simulink model "ZT_VehCtrl_18B_CAN"  (R2018b)
settings: Solver=FixedStepAuto  StartTime=0.0  StopTime=inf  FixedStep=0.005  RelTol=1e-3
InitFcn:
  | mbd_mpc_consistency_checks(bdroot(gcs));
values from neighbouring files (symbols this model uses):
  BatoverTempTh = single(80)    [VCU_INIT.m]
  BRS_PwrValid = single(5)    [VCU_INIT.m]
  BRSEnSpdTh1 = single(10)    [VCU_INIT.m]
  BRSEnSpdTh2 = single(20)    [VCU_INIT.m]
  MCUTempAlarmTh = single (60)    [VCU_INIT.m]
  mps2kmh = single(3.6)    [VCU_INIT.m]
  MtrPwrFac = single(1/9550)    [VCU_INIT.m]
  MtrTempAlarmTh = single (50)    [VCU_INIT.m]
  Padle1Signal1_Th = [PadleSignal1_min,PadleSignal1_max]    [VCU_INIT.m]
  Padle1Signal2_Th = [PadleSignal2_min,PadleSignal2_max]    [VCU_INIT.m]
  PadleSignal1_max = 3.84    [VCU_INIT.m]
  PadleSignal1_min = 0.75    [VCU_INIT.m]
  PadleSignal2_max = 1.92    [VCU_INIT.m]
  PadleSignal2_min = 0.375    [VCU_INIT.m]
  PadleValid = 0.05    [VCU_INIT.m]
  PwrLimFactor = single(0.5)    [VCU_INIT.m]
  Ratio = single(1)    [VCU_INIT.m]
  rpm2mps = single(2*pi/60 * WhlRadius/Ratio)    [VCU_INIT.m]
  SOCLowTh = single(20)    [VCU_INIT.m]
  VehPwrBackwardMax = VehPwrMax * single(0.3)    [VCU_INIT.m]
  VehPwrMax = single(MtrPwrMax * 4)    [VCU_INIT.m]
  VehTrqBackwardMax = VehTrqMax * single(0.3)    [VCU_INIT.m]
  VehTrqMax = single(MtrTrqMax * Ratio *4)    [VCU_INIT.m]
  WhlRadius = single(1)    [VCU_INIT.m]
undefined symbols (not defined in the file or in its folder): Delay_Charge, Delay_Discharge, fifo_0_vect, fifo_1_vect, LQFP, pts1_fifo_0_vect, pts1_fifo_1_vect, pts2_fifo_0_vect, pts2_fifo_1_vect, pts3_fifo_0_vect, pts3_fifo_1_vect, pts4_fifo_0_vect, pts4_fifo_1_vect
libraries: mbd_mpc574x_ec_toolbox x157, canmsglib x74, simulink x38
(part 6 of 12)

== system ZT_VehCtrl_18B_CAN/SigIn/CAN0 /BRS2VCU1 ==
  ID : Inport
  Data : Inport  Port=2
  length : Inport  Port=3
  timestamp : Inport  Port=4
  Switch Case : SwitchCase  CaseConditions={hex2dec('18FE25E4')}  ShowDefaultCase=off
  UNPACK : Subsystem  TreatAsAtomicUnit=on
  Message : Outport
  wires:
  Switch Case/1 -> UNPACK/Action
  ID/1 -> UNPACK/1(ID), Switch Case/1
  Data/1 -> UNPACK/2(data)
  timestamp/1 -> UNPACK/4(timestamp)
  length/1 -> UNPACK/3(length)
  UNPACK/1(Message) -> Message/1

== system ZT_VehCtrl_18B_CAN/SigIn/CAN0 /BRS2VCU2 ==
  ID : Inport
  Data : Inport  Port=2
  length : Inport  Port=3
  timestamp : Inport  Port=4
  Switch Case : SwitchCase  CaseConditions={hex2dec('18FE26E4')}  ShowDefaultCase=off
  UNPACK : Subsystem  TreatAsAtomicUnit=on
  Message : Outport
  wires:
  UNPACK/1(Message) -> Message/1
  length/1 -> UNPACK/3(length)
  timestamp/1 -> UNPACK/4(timestamp)
  Data/1 -> UNPACK/2(data)
  ID/1 -> Switch Case/1, UNPACK/1(ID)
  Switch Case/1 -> UNPACK/Action

== system ZT_VehCtrl_18B_CAN/SigIn/CAN0 /BRS2VCU3 ==
  ID : Inport
  Data : Inport  Port=2
  length : Inport  Port=3
  timestamp : Inport  Port=4
  Switch Case : SwitchCase  CaseConditions={hex2dec('18FE27E4')}  ShowDefaultCase=off
  UNPACK : Subsystem  TreatAsAtomicUnit=on
  Message : Outport
  wires:
  Switch Case/1 -> UNPACK/Action
  ID/1 -> UNPACK/1(ID), Switch Case/1
  Data/1 -> UNPACK/2(data)
  timestamp/1 -> UNPACK/4(timestamp)
  length/1 -> UNPACK/3(length)
  UNPACK/1(Message) -> Message/1

== system ZT_VehCtrl_18B_CAN/SigIn/CAN0 /OBC_Charger Status ==
  ID : Inport
  Data : Inport  Port=2
  length : Inport  Port=3
  timestamp : Inport  Port=4
  Switch Case : SwitchCase  CaseConditions={hex2dec('220')}  ShowDefaultCase=off
  UNPACK : Subsystem  TreatAsAtomicUnit=on
  Message : Outport
  wires:
  Switch Case/1 -> UNPACK/Action
  ID/1 -> UNPACK/1(ID), Switch Case/1
  Data/1 -> UNPACK/2(data)
  timestamp/1 -> UNPACK/4(timestamp)
  length/1 -> UNPACK/3(length)
  UNPACK/1(Message) -> Message/1

== system ZT_VehCtrl_18B_CAN/SigIn/CAN0 /PDU_RelaySts ==
  ID : Inport
  Data : Inport  Port=2
  length : Inport  Port=3
  timestamp : Inport  Port=4
  Switch Case : SwitchCase  CaseConditions={hex2dec('18FF2BC8')}  ShowDefaultCase=off
  UNPACK : Subsystem  TreatAsAtomicUnit=on
  Message : Outport
  wires:
  UNPACK/1(Message) -> Message/1
  length/1 -> UNPACK/3(length)
  timestamp/1 -> UNPACK/4(timestamp)
  Data/1 -> UNPACK/2(data)
  ID/1 -> Switch Case/1, UNPACK/1(ID)
  Switch Case/1 -> UNPACK/Action

== system ZT_VehCtrl_18B_CAN/SigIn/CAN0 /TMS2VCU ==
  ID : Inport
  Data : Inport  Port=2
  length : Inport  Port=3
  timestamp : Inport  Port=4
  Switch Case : SwitchCase  CaseConditions={hex2dec('18FFF346')}  ShowDefaultCase=off
  UNPACK : Subsystem  TreatAsAtomicUnit=on
  Message : Outport
  wires:
  UNPACK/1(Message) -> Message/1
  length/1 -> UNPACK/3(length)
  timestamp/1 -> UNPACK/4(timestamp)
  Data/1 -> UNPACK/2(data)
  ID/1 -> Switch Case/1, UNPACK/1(ID)
  Switch Case/1 -> UNPACK/Action

== system ZT_VehCtrl_18B_CAN/SigIn/CAN1/DCDC1_1 ==
  ID : Inport
  Data : Inport  Port=2
  length : Inport  Port=3
  timestamp : Inport  Port=4
  Switch Case : SwitchCase  CaseConditions={hex2dec('1800D08F')}  ShowDefaultCase=off
  UNPACK : Subsystem  TreatAsAtomicUnit=on
  Message : Outport
  wires:
  UNPACK/1(Message) -> Message/1
  length/1 -> UNPACK/3(length)
  timestamp/1 -> UNPACK/4(timestamp)
  Data/1 -> UNPACK/2(data)
  ID/1 -> Switch Case/1, UNPACK/1(ID)
  Switch Case/1 -> UNPACK/Action

== system ZT_VehCtrl_18B_CAN/SigIn/CAN1/DCDC1_2 ==
  ID : Inport
  Data : Inport  Port=2
  length : Inport  Port=3
  timestamp : Inport  Port=4
  Switch Case : SwitchCase  CaseConditions={hex2dec('1801D08F')}  ShowDefaultCase=off
  UNPACK : Subsystem  TreatAsAtomicUnit=on
  Message : Outport
  wires:
  Switch Case/1 -> UNPACK/Action
  ID/1 -> UNPACK/1(ID), Switch Case/1
  Data/1 -> UNPACK/2(data)
  timestamp/1 -> UNPACK/4(timestamp)
  length/1 -> UNPACK/3(length)
  UNPACK/1(Message) -> Message/1

== system ZT_VehCtrl_18B_CAN/SigIn/CAN1/HVC1_LV ==
  ID : Inport
  Data : Inport  Port=2
  length : Inport  Port=3
  timestamp : Inport  Port=4
  Switch Case : SwitchCase  CaseConditions={hex2dec('180105A1')}  ShowDefaultCase=off
  UNPACK : Subsystem  TreatAsAtomicUnit=on
  Message : Outport
  wires:
  Switch Case/1 -> UNPACK/Action
  ID/1 -> UNPACK/1(ID), Switch Case/1
  Data/1 -> UNPACK/2(data)
  timestamp/1 -> UNPACK/4(timestamp)
  length/1 -> UNPACK/3(length)
  UNPACK/1(Message) -> Message/1

== system ZT_VehCtrl_18B_CAN/SigIn/CAN1/HVC3_Temp ==
  ID : Inport
  Data : Inport  Port=2
  length : Inport  Port=3
  timestamp : Inport  Port=4
  Switch Case : SwitchCase  CaseConditions={hex2dec('180305A1')}  ShowDefaultCase=off
  UNPACK : Subsystem  TreatAsAtomicUnit=on
  Message : Outport
  wires:
  UNPACK/1(Message) -> Message/1
  length/1 -> UNPACK/3(length)
  timestamp/1 -> UNPACK/4(timestamp)
  Data/1 -> UNPACK/2(data)
  ID/1 -> Switch Case/1, UNPACK/1(ID)
  Switch Case/1 -> UNPACK/Action

== system ZT_VehCtrl_18B_CAN/SigIn/CAN1/HVC4_RlySt ==
  ID : Inport
  Data : Inport  Port=2
  length : Inport  Port=3
  timestamp : Inport  Port=4
  Switch Case : SwitchCase  CaseConditions={hex2dec('180405A1')}  ShowDefaultCase=off
  UNPACK : Subsystem  TreatAsAtomicUnit=on
  Message : Outport
  wires:
  Switch Case/1 -> UNPACK/Action
  ID/1 -> UNPACK/1(ID), Switch Case/1
  Data/1 -> UNPACK/2(data)
  timestamp/1 -> UNPACK/4(timestamp)
  length/1 -> UNPACK/3(length)
  UNPACK/1(Message) -> Message/1

== system ZT_VehCtrl_18B_CAN/SigIn/CAN1/HVC7_HV1 ==
  ID : Inport
  Data : Inport  Port=2
  length : Inport  Port=3
  timestamp : Inport  Port=4
  Switch Case : SwitchCase  CaseConditions={hex2dec('180705A1')}  ShowDefaultCase=off
  UNPACK : Subsystem  TreatAsAtomicUnit=on
  Message : Outport
  wires:
  UNPACK/1(Message) -> Message/1
  length/1 -> UNPACK/3(length)
  timestamp/1 -> UNPACK/4(timestamp)
  Data/1 -> UNPACK/2(data)
  ID/1 -> Switch Case/1, UNPACK/1(ID)
  Switch Case/1 -> UNPACK/Action

== system ZT_VehCtrl_18B_CAN/SigIn/CAN1/ISG MCU STATUS 1 ==
  ID : Inport
  Data : Inport  Port=2
  length : Inport  Port=3
  timestamp : Inport  Port=4
  Switch Case : SwitchCase  CaseConditions={hex2dec('CFF0006')}  ShowDefaultCase=off
  UNPACK : Subsystem  TreatAsAtomicUnit=on
  Message : Outport
  wires:
  Switch Case/1 -> UNPACK/Action
  ID/1 -> UNPACK/1(ID), Switch Case/1
  Data/1 -> UNPACK/2(data)
  timestamp/1 -> UNPACK/4(timestamp)
  length/1 -> UNPACK/3(length)
  UNPACK/1("Message ") -> Message/1

== system ZT_VehCtrl_18B_CAN/SigIn/CAN1/ISG MCU STATUS 2 ==
  ID : Inport
  Data : Inport  Port=2
  length : Inport  Port=3
  timestamp : Inport  Port=4
  Switch Case : SwitchCase  CaseConditions={hex2dec('CFF0106')}  ShowDefaultCase=off
  UNPACK : Subsystem  TreatAsAtomicUnit=on
  Message : Outport
  wires:
  UNPACK/1(Message1) -> Message/1
  length/1 -> UNPACK/3(length)
  timestamp/1 -> UNPACK/4(timestamp)
  Data/1 -> UNPACK/2(data)
  ID/1 -> Switch Case/1, UNPACK/1(ID)
  Switch Case/1 -> UNPACK/Action

== system ZT_VehCtrl_18B_CAN/SigIn/CAN1/ISG MCU STATUS 3 ==
  ID : Inport
  Data : Inport  Port=2
  length : Inport  Port=3
  timestamp : Inport  Port=4
  Switch Case : SwitchCase  CaseConditions={hex2dec('CFF0206')}  ShowDefaultCase=off
  UNPACK : Subsystem  TreatAsAtomicUnit=on
  Message : Outport
  wires:
  Switch Case/1 -> UNPACK/Action
  ID/1 -> UNPACK/1(ID), Switch Case/1
  Data/1 -> UNPACK/2(data)
  timestamp/1 -> UNPACK/4(timestamp)
  length/1 -> UNPACK/3(length)
  UNPACK/1(Message) -> Message/1

== system ZT_VehCtrl_18B_CAN/SigIn/CAN1/MCU1Msg1 ==
  ID : Inport
  Data : Inport  Port=2
  length : Inport  Port=3
  timestamp : Inport  Port=4
  Switch Case : SwitchCase  CaseConditions={hex2dec('1836D0EF')}  ShowDefaultCase=off
  UNPACK : Subsystem  TreatAsAtomicUnit=on
  Message : Outport
  wires:
  UNPACK/1(Message) -> Message/1
  length/1 -> UNPACK/3(length)
  timestamp/1 -> UNPACK/4(timestamp)
  Data/1 -> UNPACK/2(data)
  ID/1 -> Switch Case/1, UNPACK/1(ID)
  Switch Case/1 -> UNPACK/Action

== system ZT_VehCtrl_18B_CAN/SigIn/CAN1/MCU1Msg2 ==
  ID : Inport
  Data : Inport  Port=2
  length : Inport  Port=3
  timestamp : Inport  Port=4
  Switch Case : SwitchCase  CaseConditions={hex2dec('1837D0EF')}  ShowDefaultCase=off
  UNPACK : Subsystem  TreatAsAtomicUnit=on
  Message : Outport
  wires:
  Switch Case/1 -> UNPACK/Action
  ID/1 -> UNPACK/1(ID), Switch Case/1
  Data/1 -> UNPACK/2(data)
  timestamp/1 -> UNPACK/4(timestamp)
  length/1 -> UNPACK/3(length)
  UNPACK/1(Message) -> Message/1

== system ZT_VehCtrl_18B_CAN/SigIn/CAN1/MCU1Msg3 ==
  ID : Inport
  Data : Inport  Port=2
  length : Inport  Port=3
  timestamp : Inport  Port=4
  Switch Case : SwitchCase  CaseConditions={hex2dec('1838D0EF')}  ShowDefaultCase=off
  UNPACK : Subsystem  TreatAsAtomicUnit=on
  Message : Outport
  wires:
  UNPACK/1(Message) -> Message/1
  length/1 -> UNPACK/3(length)
  timestamp/1 -> UNPACK/4(timestamp)
  Data/1 -> UNPACK/2(data)
  ID/1 -> Switch Case/1, UNPACK/1(ID)
  Switch Case/1 -> UNPACK/Action

== system ZT_VehCtrl_18B_CAN/SigIn/CAN1/MCU2Msg1 ==
  ID : Inport
  Data : Inport  Port=2
  length : Inport  Port=3
  timestamp : Inport  Port=4
  Switch Case : SwitchCase  CaseConditions={hex2dec('1836D0F1')}  ShowDefaultCase=off
  UNPACK : Subsystem  TreatAsAtomicUnit=on
  Message : Outport
  wires:
  Switch Case/1 -> UNPACK/Action
  ID/1 -> UNPACK/1(ID), Switch Case/1
  Data/1 -> UNPACK/2(data)
  timestamp/1 -> UNPACK/4(timestamp)
  length/1 -> UNPACK/3(length)
  UNPACK/1(Message) -> Message/1

== system ZT_VehCtrl_18B_CAN/SigIn/CAN1/MCU2Msg2 ==
  ID : Inport
  Data : Inport  Port=2
  length : Inport  Port=3
  timestamp : Inport  Port=4
  Switch Case : SwitchCase  CaseConditions={hex2dec('1837D0F1')}  ShowDefaultCase=off
  UNPACK : Subsystem  TreatAsAtomicUnit=on
  Message : Outport
  wires:
  UNPACK/1(Message) -> Message/1
  length/1 -> UNPACK/3(length)
  timestamp/1 -> UNPACK/4(timestamp)
  Data/1 -> UNPACK/2(data)
  ID/1 -> Switch Case/1, UNPACK/1(ID)
  Switch Case/1 -> UNPACK/Action

== system ZT_VehCtrl_18B_CAN/SigIn/CAN1/MCU2Msg3 ==
  ID : Inport
  Data : Inport  Port=2
  length : Inport  Port=3
  timestamp : Inport  Port=4
  Switch Case : SwitchCase  CaseConditions={hex2dec('1838D0F1')}  ShowDefaultCase=off
  UNPACK : Subsystem  TreatAsAtomicUnit=on
  Message : Outport
  wires:
  Switch Case/1 -> UNPACK/Action
  ID/1 -> UNPACK/1(ID), Switch Case/1
  Data/1 -> UNPACK/2(data)
  timestamp/1 -> UNPACK/4(timestamp)
  length/1 -> UNPACK/3(length)
  UNPACK/1(Message) -> Message/1

== system ZT_VehCtrl_18B_CAN/SigIn/CAN1/TM MCU STATUS 1 ==
  ID : Inport
  Data : Inport  Port=2
  length : Inport  Port=3
  timestamp : Inport  Port=4
  Switch Case : SwitchCase  CaseConditions={hex2dec('CFF0005')}  ShowDefaultCase=off
  UNPACK : Subsystem  TreatAsAtomicUnit=on
  Message : Outport
  wires:
  UNPACK/1(Message) -> Message/1
  length/1 -> UNPACK/3(length)
  timestamp/1 -> UNPACK/4(timestamp)
  Data/1 -> UNPACK/2(data)
  ID/1 -> Switch Case/1, UNPACK/1(ID)
  Switch Case/1 -> UNPACK/Action

== system ZT_VehCtrl_18B_CAN/SigIn/CAN1/TM MCU STATUS 2 ==
  ID : Inport
  Data : Inport  Port=2
  length : Inport  Port=3
  timestamp : Inport  Port=4
  Switch Case : SwitchCase  CaseConditions={hex2dec('CFF0105')}  ShowDefaultCase=off
  UNPACK : Subsystem  TreatAsAtomicUnit=on
  Message : Outport
  wires:
  Switch Case/1 -> UNPACK/Action
  ID/1 -> UNPACK/1(ID), Switch Case/1
  Data/1 -> UNPACK/2(data)
  timestamp/1 -> UNPACK/4(timestamp)
  length/1 -> UNPACK/3(length)
  UNPACK/1(Message) -> Message/1

== system ZT_VehCtrl_18B_CAN/SigIn/CAN1/TM MCU STATUS 3 ==
  ID : Inport
  Data : Inport  Port=2
  length : Inport  Port=3
  timestamp : Inport  Port=4
  Switch Case : SwitchCase  CaseConditions={hex2dec('CFF0205')}  ShowDefaultCase=off
  UNPACK : Subsystem  TreatAsAtomicUnit=on
  Message : Outport
  wires:
  UNPACK/1(Message) -> Message/1
  length/1 -> UNPACK/3(length)
  timestamp/1 -> UNPACK/4(timestamp)
  Data/1 -> UNPACK/2(data)
  ID/1 -> Switch Case/1, UNPACK/1(ID)
  Switch Case/1 -> UNPACK/Action

== system ZT_VehCtrl_18B_CAN/SigIn/CAN1/TWV  ==
  ID : Inport
  Data : Inport  Port=2
  length : Inport  Port=3
  timestamp : Inport  Port=4
  Switch Case : SwitchCase  CaseConditions={hex2dec('18FF243B')}  ShowDefaultCase=off
  UNPACK : Subsystem  TreatAsAtomicUnit=on
  Message : Outport
  wires:
  Switch Case/1 -> UNPACK/Action
  ID/1 -> UNPACK/1(ID), Switch Case/1
  Data/1 -> UNPACK/2(data)
  timestamp/1 -> UNPACK/4(timestamp)
  length/1 -> UNPACK/3(length)
  UNPACK/1(Message) -> Message/1

== system ZT_VehCtrl_18B_CAN/SigIn/DI/DI_31_32_33_34 ==
  note: DI PWM PULLUP
  note: DI PWM PULLDOWN
  DI31 : mbd_mpc574x_ec_toolbox/GPIO Blocks/Digital_Input  gpio_pin=PTF0: [SIUL2_GPIO80 | General Purpose IO PF[0]]  pull_resistor=None
  DI32 : mbd_mpc574x_ec_toolbox/GPIO Blocks/Digital_Input  gpio_pin=PTD1: [SIUL2_GPIO49 | General Purpose IO PD[1]]  pull_resistor=None
  DI33 : mbd_mpc574x_ec_toolbox/GPIO Blocks/Digital_Input  gpio_pin=PTD2: [SIUL2_GPIO50 | General Purpose IO PD[2]]  pull_resistor=None
  DI34 : mbd_mpc574x_ec_toolbox/GPIO Blocks/Digital_Input  gpio_pin=PTC13: [SIUL2_GPIO45 | General Purpose IO PC[13]]  pull_resistor=None
  Data Store Write14 : DataStoreWrite  DataStoreName=DI31
  Data Store Write15 : DataStoreWrite  DataStoreName=DI32
  Data Store Write16 : DataStoreWrite  DataStoreName=DI33
  Data Store Write17 : DataStoreWrite  DataStoreName=DI34
  wires:
  DI34/1 -> Data Store Write17/1
  DI33/1 -> Data Store Write16/1
  DI32/1 -> Data Store Write15/1
  DI31/1 -> Data Store Write14/1

== system ZT_VehCtrl_18B_CAN/SigIn/PWM/PWM_PTS1 ==
  Add : Sum  Inputs=+-  AccumDataTypeStr=single
  Add1 : Sum  Inputs=+-  AccumDataTypeStr=single
  Data Store Memory : DataStoreMemory  DataStoreName=pts1_pwm_cnt  ReadBeforeWriteMsg=warning  WriteAfterWriteMsg=warning  WriteAfterReadMsg=warning  ShowAdditionalParam=off  OutDataTypeStr=uint8
  Data Store Memory2 : DataStoreMemory  DataStoreName=pts1_fifo_1_vect  ReadBeforeWriteMsg=warning  WriteAfterWriteMsg=warning  WriteAfterReadMsg=warning  InitialValue=[0 0 0 0 0 0 0 0]  ShowAdditionalParam=off  OutDataTypeStr=uint16
  Data Store Memory4 : DataStoreMemory  DataStoreName=pts1_fifo_0_vect  ReadBeforeWriteMsg=warning  WriteAfterWriteMsg=warning  WriteAfterReadMsg=warning  InitialValue=[0 0 0 0 0 0 0 0]  ShowAdditionalParam=off  OutDataTypeStr=uint16
  Data Store Read : DataStoreRead  DataStoreName=pts1_fifo_0_vect  DataStoreElements=pts1_fifo_0_vect(2)#pts1_fifo_0_vect(1)
  Data Store Read1 : DataStoreRead  DataStoreName=pts1_fifo_1_vect  DataStoreElements=pts1_fifo_1_vect(1)
  Data Store Read2 : DataStoreRead  DataStoreName=pts1_fifo_0_vect  DataStoreElements=pts1_fifo_0_vect(1)
  Data Store Write3 : DataStoreWrite  DataStoreName=pts1_fifo_0_vect
  Data Store Write5 : DataStoreWrite  DataStoreName=pts1_fifo_1_vect
  Divide : Product  Inputs=*/  OutDataTypeStr=single
  Divide1 : Product  Inputs=*//
  Freq_MC : Constant  Value=80000000  OutDataTypeStr=single
  Prescaler : Constant  Value=32  OutDataTypeStr=single
  Subsystem : Subsystem
  Subsystem_capture : Subsystem
  Terminator1 : Terminator
  Terminator2 : Terminator
  eTimer_ISR : mbd_mpc574x_ec_toolbox/Motor Control Blocks/eTIMER Blocks/eTimer_ISR_Handler  etimerModule=1  etimerInterrupt=Channel Interrupt  etimerChannel=2  etimerIsrPriority=14
      settings: SourceProductName=NXP Model-Based Design Toolbox for MPC57xx MCUs
  DC : Outport
  freq : Outport  Port=2
  wires:
  eTimer_ISR/2 -> Subsystem_capture/1(In1)
  Subsystem_capture/1(Out1) -> Terminator1/1
  Subsystem_capture/3(Out3) -> Terminator2/1
  Subsystem_capture/4(Out4) -> Data Store Write5/1
  Subsystem_capture/2(Out2) -> Data Store Write3/1
  eTimer_ISR/1 -> Subsystem_capture/Trigger
  Prescaler/1 -> Divide1/2
  Add/1 -> Divide/2, Divide1/3
  Data Store Read1/1 -> Add1/1
  Data Store Read/2 -> Add/2
  Freq_MC/1 -> Divide1/1
  Add1/1 -> Divide/1
  Data Store Read2/1 -> Add1/2
  Divide1/1 -> freq/1
  Data Store Read/1 -> Add/1
  Divide/1 -> Subsystem/1(In1)
  Subsystem/1(Out1) -> DC/1

== system ZT_VehCtrl_18B_CAN/SigIn/PWM/PWM_PTS2 ==
  Add : Sum  Inputs=+-  AccumDataTypeStr=single
  Add1 : Sum  Inputs=+-  AccumDataTypeStr=single
  Data Store Memory : DataStoreMemory  DataStoreName=pts2_pwm_cnt  ReadBeforeWriteMsg=warning  WriteAfterWriteMsg=warning  WriteAfterReadMsg=warning  ShowAdditionalParam=off  OutDataTypeStr=uint8
  Data Store Memory2 : DataStoreMemory  DataStoreName=pts2_fifo_1_vect  ReadBeforeWriteMsg=warning  WriteAfterWriteMsg=warning  WriteAfterReadMsg=warning  InitialValue=[0 0 0 0 0 0 0 0]  ShowAdditionalParam=off  OutDataTypeStr=uint16
  Data Store Memory4 : DataStoreMemory  DataStoreName=pts2_fifo_0_vect  ReadBeforeWriteMsg=warning  WriteAfterWriteMsg=warning  WriteAfterReadMsg=warning  InitialValue=[0 0 0 0 0 0 0 0]  ShowAdditionalParam=off  OutDataTypeStr=uint16
  Data Store Read : DataStoreRead  DataStoreName=pts2_fifo_0_vect  DataStoreElements=pts2_fifo_0_vect(2)#pts2_fifo_0_vect(1)
  Data Store Read1 : DataStoreRead  DataStoreName=pts2_fifo_1_vect  DataStoreElements=pts2_fifo_1_vect(1)
  Data Store Read2 : DataStoreRead  DataStoreName=pts2_fifo_0_vect  DataStoreElements=pts2_fifo_0_vect(1)
  Data Store Write3 : DataStoreWrite  DataStoreName=pts2_fifo_0_vect
  Data Store Write5 : DataStoreWrite  DataStoreName=pts2_fifo_1_vect
  Divide : Product  Inputs=*/  OutDataTypeStr=single
  Divide1 : Product  Inputs=*//
  Freq_MC : Constant  Value=80000000  OutDataTypeStr=single
  Prescaler : Constant  Value=32  OutDataTypeStr=single
  Subsystem : Subsystem
  Subsystem_capture : Subsystem
  Terminator1 : Terminator
  Terminator2 : Terminator
  eTimer_ISR : mbd_mpc574x_ec_toolbox/Motor Control Blocks/eTIMER Blocks/eTimer_ISR_Handler  etimerModule=1  etimerInterrupt=Channel Interrupt  etimerChannel=3  etimerIsrPriority=14
      settings: SourceProductName=NXP Model-Based Design Toolbox for MPC57xx MCUs
  DC : Outport
  freq : Outport  Port=2
  wires:
  Subsystem/1(Out1) -> DC/1
  Divide/1 -> Subsystem/1(In1)
  Data Store Read/1 -> Add/1
  Divide1/1 -> freq/1
  Data Store Read2/1 -> Add1/2
  Add1/1 -> Divide/1
  Freq_MC/1 -> Divide1/1
  Data Store Read/2 -> Add/2
  Data Store Read1/1 -> Add1/1
  Add/1 -> Divide1/3, Divide/2
  Prescaler/1 -> Divide1/2
  eTimer_ISR/1 -> Subsystem_capture/Trigger
  Subsystem_capture/2(Out2) -> Data Store Write3/1
  Subsystem_capture/4(Out4) -> Data Store Write5/1
  Subsystem_capture/3(Out3) -> Terminator2/1
  Subsystem_capture/1(Out1) -> Terminator1/1
  eTimer_ISR/2 -> Subsystem_capture/1(In1)

== system ZT_VehCtrl_18B_CAN/SigIn/PWM/PWM_PTS3 ==
  Add : Sum  Inputs=+-  AccumDataTypeStr=single
  Add1 : Sum  Inputs=+-  AccumDataTypeStr=single
  Data Store Memory : DataStoreMemory  DataStoreName=pts3_pwm_cnt  ReadBeforeWriteMsg=warning  WriteAfterWriteMsg=warning  WriteAfterReadMsg=warning  ShowAdditionalParam=off  OutDataTypeStr=uint8
  Data Store Memory2 : DataStoreMemory  DataStoreName=pts3_fifo_1_vect  ReadBeforeWriteMsg=warning  WriteAfterWriteMsg=warning  WriteAfterReadMsg=warning  InitialValue=[0 0 0 0 0 0 0 0]  ShowAdditionalParam=off  OutDataTypeStr=uint16
  Data Store Memory4 : DataStoreMemory  DataStoreName=pts3_fifo_0_vect  ReadBeforeWriteMsg=warning  WriteAfterWriteMsg=warning  WriteAfterReadMsg=warning  InitialValue=[0 0 0 0 0 0 0 0]  ShowAdditionalParam=off  OutDataTypeStr=uint16
  Data Store Read : DataStoreRead  DataStoreName=pts3_fifo_0_vect  DataStoreElements=pts3_fifo_0_vect(2)#pts3_fifo_0_vect(1)
  Data Store Read1 : DataStoreRead  DataStoreName=pts3_fifo_1_vect  DataStoreElements=pts3_fifo_1_vect(1)
  Data Store Read2 : DataStoreRead  DataStoreName=pts3_fifo_0_vect  DataStoreElements=pts3_fifo_0_vect(1)
  Data Store Write3 : DataStoreWrite  DataStoreName=pts3_fifo_0_vect
  Data Store Write5 : DataStoreWrite  DataStoreName=pts3_fifo_1_vect
  Divide : Product  Inputs=*/  OutDataTypeStr=single
  Divide1 : Product  Inputs=*//
  Freq_MC : Constant  Value=80000000  OutDataTypeStr=single
  Prescaler : Constant  Value=32  OutDataTypeStr=single
  Subsystem : Subsystem
  Subsystem_capture : Subsystem
  Terminator1 : Terminator
  Terminator2 : Terminator
  eTimer_ISR : mbd_mpc574x_ec_toolbox/Motor Control Blocks/eTIMER Blocks/eTimer_ISR_Handler  etimerModule=1  etimerInterrupt=Channel Interrupt  etimerChannel=1  etimerIsrPriority=14
      settings: SourceProductName=NXP Model-Based Design Toolbox for MPC57xx MCUs
  DC : Outport
  freq : Outport  Port=2
  wires:
  eTimer_ISR/2 -> Subsystem_capture/1(In1)
  Subsystem_capture/1(Out1) -> Terminator1/1
  Subsystem_capture/3(Out3) -> Terminator2/1
  Subsystem_capture/4(Out4) -> Data Store Write5/1
  Subsystem_capture/2(Out2) -> Data Store Write3/1
  eTimer_ISR/1 -> Subsystem_capture/Trigger
  Prescaler/1 -> Divide1/2
  Add/1 -> Divide/2, Divide1/3
  Data Store Read1/1 -> Add1/1
  Data Store Read/2 -> Add/2
  Freq_MC/1 -> Divide1/1
  Add1/1 -> Divide/1
  Data Store Read2/1 -> Add1/2
  Divide1/1 -> freq/1
  Data Store Read/1 -> Add/1
  Divide/1 -> Subsystem/1(In1)
  Subsystem/1(Out1) -> DC/1

== system ZT_VehCtrl_18B_CAN/SigIn/PWM/PWM_PTS4 ==
  Add : Sum  Inputs=+-  AccumDataTypeStr=single
  Add1 : Sum  Inputs=+-  AccumDataTypeStr=single
  Data Store Memory : DataStoreMemory  DataStoreName=pts4_pwm_cnt  ReadBeforeWriteMsg=warning  WriteAfterWriteMsg=warning  WriteAfterReadMsg=warning  ShowAdditionalParam=off  OutDataTypeStr=uint8
  Data Store Memory2 : DataStoreMemory  DataStoreName=pts4_fifo_1_vect  ReadBeforeWriteMsg=warning  WriteAfterWriteMsg=warning  WriteAfterReadMsg=warning  InitialValue=[0 0 0 0 0 0 0 0]  ShowAdditionalParam=off  OutDataTypeStr=uint16
  Data Store Memory4 : DataStoreMemory  DataStoreName=pts4_fifo_0_vect  ReadBeforeWriteMsg=warning  WriteAfterWriteMsg=warning  WriteAfterReadMsg=warning  InitialValue=[0 0 0 0 0 0 0 0]  ShowAdditionalParam=off  OutDataTypeStr=uint16
  Data Store Read : DataStoreRead  DataStoreName=pts4_fifo_0_vect  DataStoreElements=pts4_fifo_0_vect(2)#pts4_fifo_0_vect(1)
  Data Store Read1 : DataStoreRead  DataStoreName=pts4_fifo_1_vect  DataStoreElements=pts4_fifo_1_vect(1)
  Data Store Read2 : DataStoreRead  DataStoreName=pts4_fifo_0_vect  DataStoreElements=pts4_fifo_0_vect(1)
  Data Store Write3 : DataStoreWrite  DataStoreName=pts4_fifo_0_vect
  Data Store Write5 : DataStoreWrite  DataStoreName=pts4_fifo_1_vect
  Divide : Product  Inputs=*/  OutDataTypeStr=single
  Divide1 : Product  Inputs=*//
  Freq_MC : Constant  Value=80000000  OutDataTypeStr=single
  Prescaler : Constant  Value=32  OutDataTypeStr=single
  Subsystem : Subsystem
  Subsystem_capture : Subsystem
  Terminator1 : Terminator
  Terminator2 : Terminator
  eTimer_ISR : mbd_mpc574x_ec_toolbox/Motor Control Blocks/eTIMER Blocks/eTimer_ISR_Handler  etimerModule=0  etimerInterrupt=Channel Interrupt  etimerChannel=2  etimerIsrPriority=14
      settings: SourceProductName=NXP Model-Based Design Toolbox for MPC57xx MCUs
  DC : Outport
  freq : Outport  Port=2
  wires:
  Subsystem/1(Out1) -> DC/1
  Divide/1 -> Subsystem/1(In1)
  Data Store Read/1 -> Add/1
  Divide1/1 -> freq/1
  Data Store Read2/1 -> Add1/2
  Add1/1 -> Divide/1
  Freq_MC/1 -> Divide1/1
  Data Store Read/2 -> Add/2
  Data Store Read1/1 -> Add1/1
  Add/1 -> Divide1/3, Divide/2
  Prescaler/1 -> Divide1/2
  eTimer_ISR/1 -> Subsystem_capture/Trigger
  Subsystem_capture/2(Out2) -> Data Store Write3/1
  Subsystem_capture/4(Out4) -> Data Store Write5/1
  Subsystem_capture/3(Out3) -> Terminator2/1
  Subsystem_capture/1(Out1) -> Terminator1/1
  eTimer_ISR/2 -> Subsystem_capture/1(In1)

== system ZT_VehCtrl_18B_CAN/SigIn/PWM/Subsystem ==
  Data Store Memory1 : DataStoreMemory  DataStoreName=fifo_1_value  ReadBeforeWriteMsg=warning  WriteAfterWriteMsg=warning  WriteAfterReadMsg=warning  VectorParams1D=off  ShowAdditionalParam=off  OutDataTypeStr=uint16
  Data Store Memory3 : DataStoreMemory  DataStoreName=fifo_0_value  ReadBeforeWriteMsg=warning  WriteAfterWriteMsg=warning  WriteAfterReadMsg=warning  VectorParams1D=off  ShowAdditionalParam=off  OutDataTypeStr=uint16
  Data Store Memory5 : DataStoreMemory  DataStoreName=frequency  ReadBeforeWriteMsg=warning  WriteAfterWriteMsg=warning  WriteAfterReadMsg=warning  VectorParams1D=off  ShowAdditionalParam=off  OutDataTypeStr=single
  Data Store Memory6 : DataStoreMemory  DataStoreName=duty_cycle  ReadBeforeWriteMsg=warning  WriteAfterWriteMsg=warning  WriteAfterReadMsg=warning  VectorParams1D=off  ShowAdditionalParam=off  OutDataTypeStr=single
  Data Store Write10 : DataStoreWrite  DataStoreName=fifo_0_vect
  Data Store Write11 : DataStoreWrite  DataStoreName=fifo_1_value
  Data Store Write12 : DataStoreWrite  DataStoreName=fifo_1_vect
  Data Store Write13 : DataStoreWrite  DataStoreName=duty_cycle
  Data Store Write8 : DataStoreWrite  DataStoreName=frequency
  Data Store Write9 : DataStoreWrite  DataStoreName=fifo_0_value
  Frequency_DutyCycle_Computation : Subsystem
  eTimer Configuration and Signal Measurements : Subsystem
  wires:
  eTimer Configuration and Signal Measurements/4(Out4) -> Data Store Write12/1
  eTimer Configuration and Signal Measurements/2(Out2) -> Data Store Write10/1
  eTimer Configuration and Signal Measurements/3(Out3) -> Data Store Write11/1
  eTimer Configuration and Signal Measurements/1(Out1) -> Data Store Write9/1
  Frequency_DutyCycle_Computation/2(Out2) -> Data Store Write8/1
  Frequency_DutyCycle_Computation/1(Out1) -> Data Store Write13/1

== system ZT_VehCtrl_18B_CAN/SigOut/ACU/Subsystem1 ==
  <DcacEpsCmd> : Inport
  Constant1 : Constant  Value=85  OutDataTypeStr=single
  Constant2 : Constant  Value=170  OutDataTypeStr=single
  Switch : Switch  Criteria=u2 > Threshold
  Out1 : Outport
  wires:
  Constant2/1 -> Switch/3
  Constant1/1 -> Switch/1
  Switch/1 -> Out1/1
  <DcacEpsCmd>/1 -> Switch/2

== system ZT_VehCtrl_18B_CAN/SigOut/ACU/Subsystem2 ==
  <DcacEpsCmd> : Inport
  Constant1 : Constant  Value=85  OutDataTypeStr=single
  Constant2 : Constant  Value=170  OutDataTypeStr=single
  Switch : Switch  Criteria=u2 > Threshold
  Out1 : Outport
  wires:
  <DcacEpsCmd>/1 -> Switch/2
  Switch/1 -> Out1/1
  Constant1/1 -> Switch/1
  Constant2/1 -> Switch/3

== system ZT_VehCtrl_18B_CAN/SigOut/ACU/Subsystem3 ==
  <DcacEpsCmd> : Inport
  Constant1 : Constant  Value=85  OutDataTypeStr=single
  Constant2 : Constant  Value=170  OutDataTypeStr=single
  Switch : Switch  Criteria=u2 > Threshold
  Out1 : Outport
  wires:
  <DcacEpsCmd>/1 -> Switch/2
  Switch/1 -> Out1/1
  Constant1/1 -> Switch/1
  Constant2/1 -> Switch/3

== system ZT_VehCtrl_18B_CAN/SigOut/ACU/Subsystem4 ==
  <DcacEpsCmd> : Inport
  Constant1 : Constant  Value=85  OutDataTypeStr=single
  Constant2 : Constant  Value=170  OutDataTypeStr=single
  Switch : Switch  Criteria=u2 > Threshold
  Out1 : Outport
  wires:
  Constant2/1 -> Switch/3
  Constant1/1 -> Switch/1
  Switch/1 -> Out1/1
  <DcacEpsCmd>/1 -> Switch/2

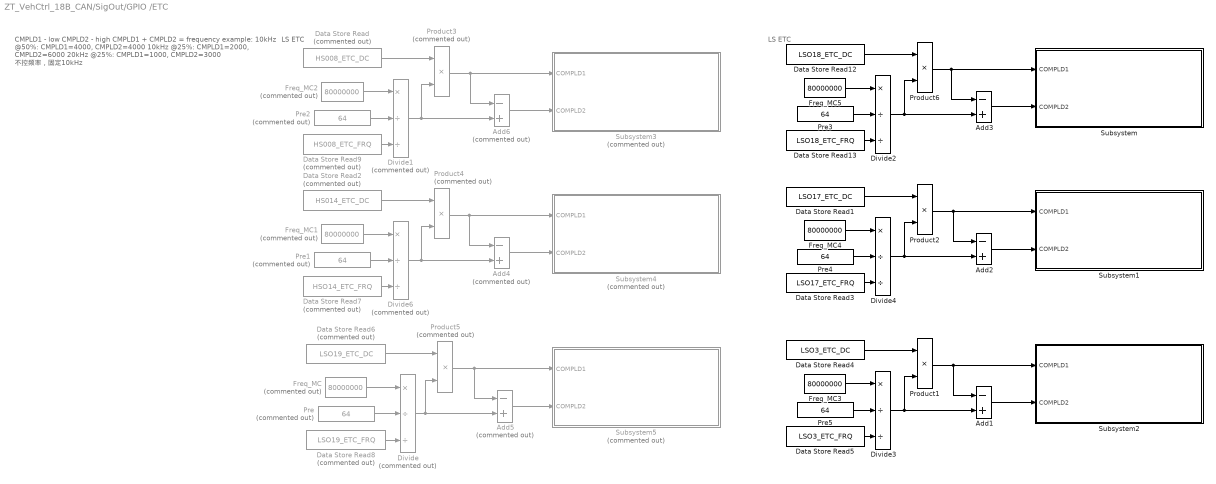
== system ZT_VehCtrl_18B_CAN/SigOut/GPIO /ETC ==
  note: CMPLD1 - low
      | CMPLD2 - high
      | CMPLD1 + CMPLD2 = frequency
      | example:
      | 10kHz @50%: CMPLD1=4000, CMPLD2=4000
      | 10kHz @25%: CMPLD1=2000, CMPLD2=6000
      | 20kHz @25%: CMPLD1=1000, CMPLD2=3000
      |
      | 不控频率，固定10kHz
  note: LS ETC
  note: LS ETC
  Add1 : Sum  Inputs=-+
  Add2 : Sum  Inputs=-+
  Add3 : Sum  Inputs=-+
  Add4 : Sum  Commented=on  Inputs=-+
  Add5 : Sum  Commented=on  Inputs=-+
  Add6 : Sum  Commented=on  Inputs=-+
  Data Store Read : DataStoreRead  Commented=on  DataStoreName=HS008_ETC_DC
  Data Store Read1 : DataStoreRead  DataStoreName=LSO17_ETC_DC
  Data Store Read12 : DataStoreRead  DataStoreName=LSO18_ETC_DC
  Data Store Read13 : DataStoreRead  DataStoreName=LSO18_ETC_FRQ
  Data Store Read2 : DataStoreRead  Commented=on  DataStoreName=HS014_ETC_DC
  Data Store Read3 : DataStoreRead  DataStoreName=LSO17_ETC_FRQ
  Data Store Read4 : DataStoreRead  DataStoreName=LSO3_ETC_DC
  Data Store Read5 : DataStoreRead  DataStoreName=LSO3_ETC_FRQ
  Data Store Read6 : DataStoreRead  Commented=on  DataStoreName=LSO19_ETC_DC
  Data Store Read7 : DataStoreRead  Commented=on  DataStoreName=HSO14_ETC_FRQ
  Data Store Read8 : DataStoreRead  Commented=on  DataStoreName=LSO19_ETC_FRQ
  Data Store Read9 : DataStoreRead  Commented=on  DataStoreName=HS008_ETC_FRQ
  Divide : Product  Commented=on  Inputs=*//
  Divide1 : Product  Commented=on  Inputs=*//
  Divide2 : Product  Inputs=*//
  Divide3 : Product  Inputs=*//
  Divide4 : Product  Inputs=*//
  Divide6 : Product  Commented=on  Inputs=*//
  Freq_MC : Constant  Commented=on  Value=80000000  OutDataTypeStr=single
  Freq_MC1 : Constant  Commented=on  Value=80000000  OutDataTypeStr=single
  Freq_MC2 : Constant  Commented=on  Value=80000000  OutDataTypeStr=single
  Freq_MC3 : Constant  Value=80000000  OutDataTypeStr=single
  Freq_MC4 : Constant  Value=80000000  OutDataTypeStr=single
  Freq_MC5 : Constant  Value=80000000  OutDataTypeStr=single
  Pre : Constant  Commented=on  Value=64
  Pre1 : Constant  Commented=on  Value=64
  Pre2 : Constant  Commented=on  Value=64
  Pre3 : Constant  Value=64
  Pre4 : Constant  Value=64
  Pre5 : Constant  Value=64
  Product1 : Product
  Product2 : Product
  Product3 : Product  Commented=on
  Product4 : Product  Commented=on
  Product5 : Product  Commented=on
  Product6 : Product
  Subsystem : Subsystem
  Subsystem1 : Subsystem
  Subsystem2 : Subsystem
  Subsystem3 : Subsystem  Commented=on
  Subsystem4 : Subsystem  Commented=on
  Subsystem5 : Subsystem  Commented=on
  wires:
  Data Store Read6/1 -> Product5/1
  Product5/1 -> Add5/1, Subsystem5/1(COMPLD1)
  Add5/1 -> Subsystem5/2(COMPLD2)
  Add4/1 -> Subsystem4/2(COMPLD2)
  Data Store Read8/1 -> Divide/3
  Data Store Read2/1 -> Product4/1
  Freq_MC/1 -> Divide/1
  Divide/1 -> Product5/2, Add5/2
  Divide6/1 -> Product4/2, Add4/2
  Freq_MC1/1 -> Divide6/1
  Data Store Read7/1 -> Divide6/3
  Product4/1 -> Add4/1, Subsystem4/1(COMPLD1)
  Divide1/1 -> Product3/2, Add6/2
  Freq_MC2/1 -> Divide1/1
  Data Store Read9/1 -> Divide1/3
  Product3/1 -> Add6/1, Subsystem3/1(COMPLD1)
  Data Store Read/1 -> Product3/1
  Add6/1 -> Subsystem3/2(COMPLD2)
  Divide3/1 -> Product1/2, Add1/2
  Freq_MC3/1 -> Divide3/1
  Data Store Read5/1 -> Divide3/3
  Product1/1 -> Add1/1, Subsystem2/1(COMPLD1)
  Divide4/1 -> Product2/2, Add2/2
  Freq_MC4/1 -> Divide4/1
  Data Store Read3/1 -> Divide4/3
  Product2/1 -> Add2/1, Subsystem1/1(COMPLD1)
  Divide2/1 -> Product6/2, Add3/2
  Freq_MC5/1 -> Divide2/1
  Data Store Read13/1 -> Divide2/3
  Product6/1 -> Add3/1, Subsystem/1(COMPLD1)
  Data Store Read1/1 -> Product2/1
  Data Store Read4/1 -> Product1/1
  Data Store Read12/1 -> Product6/1
  Add1/1 -> Subsystem2/2(COMPLD2)
  Add2/1 -> Subsystem1/2(COMPLD2)
  Add3/1 -> Subsystem/2(COMPLD2)
  Pre/1 -> Divide/2
  Pre1/1 -> Divide6/2
  Pre2/1 -> Divide1/2
  Pre3/1 -> Divide2/2
  Pre4/1 -> Divide4/2
  Pre5/1 -> Divide3/2

== system ZT_VehCtrl_18B_CAN/SigOut/GPIO /HS ==
  note: 3A/5A
  note: 1A/3A
  note: 0.5A/1A
  Data Store Read : DataStoreRead  DataStoreName=HS001
  Data Store Read2 : DataStoreRead  DataStoreName=HS007
  Data Store Read4 : DataStoreRead  DataStoreName=HS002
  Data Store Read5 : DataStoreRead  DataStoreName=HS003
  Data Store Read6 : DataStoreRead  DataStoreName=HS004
  Data Store Read7 : DataStoreRead  DataStoreName=HS005
  Data Store Read9 : DataStoreRead  DataStoreName=HS010
  HS001 : mbd_mpc574x_ec_toolbox/GPIO Blocks/Digital_Output  Priority=1  gpio_pin=PTF5: [SIUL2_GPIO85 | General Purpose IO PF[5]]  gpio_drive_strength=Disabled
  "HS002 " : mbd_mpc574x_ec_toolbox/GPIO Blocks/Digital_Output  Priority=1  gpio_pin=PTF4: [SIUL2_GPIO84 | General Purpose IO PF[4]]  gpio_drive_strength=Disabled
  HS003 : mbd_mpc574x_ec_toolbox/GPIO Blocks/Digital_Output  Priority=1  gpio_pin=PTF3: [SIUL2_GPIO83 | General Purpose IO PF[3]]  gpio_drive_strength=Disabled
  HS004 : mbd_mpc574x_ec_toolbox/GPIO Blocks/Digital_Output  Priority=1  gpio_pin=PTB6: [SIUL2_GPIO22 | General Purpose IO PB[6]]  gpio_drive_strength=Disabled
  HS005 : mbd_mpc574x_ec_toolbox/GPIO Blocks/Digital_Output  Priority=1  gpio_pin=PTA12: [SIUL2_GPIO12 | General Purpose IO PA[12]]  gpio_drive_strength=Disabled
  HS007 : mbd_mpc574x_ec_toolbox/GPIO Blocks/Digital_Output  Priority=1  gpio_pin=PTF7: [SIUL2_GPIO87 | General Purpose IO PF[7]]  gpio_drive_strength=Disabled
  HS010 : mbd_mpc574x_ec_toolbox/GPIO Blocks/Digital_Output  Priority=1  gpio_pin=PTF9: [SIUL2_GPIO89 | General Purpose IO PF[9]]  gpio_drive_strength=Disabled
  wires:
  Data Store Read/1 -> HS001/1
  Data Store Read5/1 -> HS003/1
  Data Store Read4/1 -> "HS002 "/1
  Data Store Read6/1 -> HS004/1
  Data Store Read7/1 -> HS005/1
  Data Store Read2/1 -> HS007/1
  Data Store Read9/1 -> HS010/1

== system ZT_VehCtrl_18B_CAN/SigOut/GPIO /PWM_OUT ==
  note: LS PWM
  note: HS PWM
  note: Example
  Data Store Read10 : DataStoreRead  DataStoreName=HSO14_PWM_DC
  Data Store Read11 : DataStoreRead  DataStoreName=HSO14_PWM_FRQ
  Data Store Read14 : DataStoreRead  DataStoreName=LSO19_PWM_DC
  Data Store Read15 : DataStoreRead  DataStoreName=LSO19_PWM_FRQ
  Data Store Read2 : DataStoreRead  DataStoreName=HSO08_PWM_DC
  Data Store Read9 : DataStoreRead  DataStoreName=HSO08_PWM_FRQ
  FreqCMD : Stateflow chart  Priority=0  Commented=on  TreatAsAtomicUnit=on
  PWM Configuration and Frequency Update : Subsystem  Commented=on
  PWM Configuration and Frequency Update1 : Subsystem
  PWM Configuration and Frequency Update4 : Subsystem
  wires:
  FreqCMD/1(freq) -> PWM Configuration and Frequency Update/1(In1)
  FreqCMD/2(dc) -> PWM Configuration and Frequency Update/2(In2)
  Data Store Read9/1 -> PWM Configuration and Frequency Update1/2(Fre A)
  Data Store Read2/1 -> PWM Configuration and Frequency Update1/1(PWM A)
  Data Store Read14/1 -> PWM Configuration and Frequency Update4/1(PWM A)
  Data Store Read10/1 -> PWM Configuration and Frequency Update1/3(PWM B)
  Data Store Read11/1 -> PWM Configuration and Frequency Update1/4(Fre B)
  Data Store Read15/1 -> PWM Configuration and Frequency Update4/2(Fre)

== system ZT_VehCtrl_18B_CAN/SigOut/GPIO /SPI0: LS09_14_15_16_1_2_11_4 ==
  note: 不要开，会重置SPI的初始化设置
  Compare To Constant : simulink/Logic and Bit Operations/Compare To Constant  relop===  const=2  OutDataTypeStr=boolean
  Constant : Constant  OutDataTypeStr=boolean
  Constant1 : Constant  OutDataTypeStr=boolean
  Constant2 : Constant  OutDataTypeStr=boolean
  Data Store Read : DataStoreRead  DataStoreName=VCU_Mode
  Data Store Read1 : DataStoreRead  DataStoreName=SPI0_CS
  LS_CTRL : Subsystem
  LS_CTRL1 : Subsystem
  LS_EN : mbd_mpc574x_ec_toolbox/GPIO Blocks/Digital_Output  Priority=1  gpio_pin=PTA2: [SIUL2_GPIO2 | General Purpose IO PA[2]]  gpio_drive_strength=Disabled
  LS_rst1 : mbd_mpc574x_ec_toolbox/GPIO Blocks/Digital_Output  Priority=1  gpio_pin=PTC10: [SIUL2_GPIO42 | General Purpose IO PC[10]]  gpio_drive_strength=Disabled
  LS_rst2 : mbd_mpc574x_ec_toolbox/GPIO Blocks/Digital_Output  Priority=1  gpio_pin=PTA1: [SIUL2_GPIO1 | General Purpose IO PA[1]]  gpio_drive_strength=Disabled
  Logical Operator : Logic  AllPortsSameDT=off  OutDataTypeStr=boolean
  Logical Operator1 : Logic  Operator=NOT  AllPortsSameDT=off  OutDataTypeStr=boolean
  wires:
  Constant1/1 -> LS_rst2/1
  Constant/1 -> LS_EN/1
  Constant2/1 -> LS_rst1/1
  Data Store Read/1 -> Compare To Constant/1
  Compare To Constant/1 -> Logical Operator/1
  Data Store Read1/1 -> Logical Operator/2
  Logical Operator/1 -> LS_CTRL1/Enable, Logical Operator1/1
  Logical Operator1/1 -> LS_CTRL/Enable

== system ZT_VehCtrl_18B_CAN/SigOut/GPIO /SPI3: LS03_06_07_08_10_12_13_17_18_19 ==
  Compare To Constant : simulink/Logic and Bit Operations/Compare To Constant  relop===  const=2  OutDataTypeStr=boolean
  Constant1 : Constant  OutDataTypeStr=boolean
  Constant3 : Constant  OutDataTypeStr=boolean
  Data Store Read : DataStoreRead  DataStoreName=VCU_Mode
  Data Store Read3 : DataStoreRead  DataStoreName=SPI3_CS
  LS_EN1 : mbd_mpc574x_ec_toolbox/GPIO Blocks/Digital_Output  Priority=1  gpio_pin=PTF10: [SIUL2_GPIO90 | General Purpose IO PF[10]]  gpio_drive_strength=Disabled
  LS_rst : mbd_mpc574x_ec_toolbox/GPIO Blocks/Digital_Output  Priority=1  gpio_pin=PTC14: [SIUL2_GPIO46 | General Purpose IO PC[14]]  gpio_drive_strength=Disabled
  Logical Operator : Logic  AllPortsSameDT=off  OutDataTypeStr=boolean
  Subsystem : Subsystem
  wires:
  Constant1/1 -> LS_EN1/1
  Constant3/1 -> LS_rst/1
  Data Store Read/1 -> Compare To Constant/1
  Data Store Read3/1 -> Logical Operator/2
  Compare To Constant/1 -> Logical Operator/1
  Logical Operator/1 -> Subsystem/Enable

== system ZT_VehCtrl_18B_CAN/VehCtrl/MontionControl/VehTrqBackward ==
  VehSpd : Inport
  VehDrvPct : Inport  Port=2
  PwrLim : Inport  Port=3
  Abs : Abs
  Constant : Constant  Value=VehTrqBackwardMax
  Constant1 : Constant  Value=VehPwrBackwardMax
  Constant2 : Constant  Value=WhlRadius
  Constant3 : Constant  Value=0.1  OutDataTypeStr=single
  Divide : Product  Inputs=*/
  Divide1 : Product  Inputs=*/
  Gain : Gain  Gain=1000
  Gain2 : Gain  Gain=PwrLimFactor
  Max : MinMax  Function=max  Inputs=2
  Min : MinMax  Inputs=2
  Product : Product
  Product1 : Product
  Product2 : Product
  Switch : Switch  Criteria=u2 > Threshold
  VehTrq : Outport
  wires:
  Constant/1 -> Product1/2
  Product1/1 -> Min/1
  VehDrvPct/1 -> Product/2, Product/1, Product1/1
  Product2/1 -> Divide/1
  Divide1/1 -> Divide/2
  Product/1 -> Product2/1
  Divide/1 -> Min/2
  Min/1 -> VehTrq/1
  Constant2/1 -> Divide1/2
  Constant3/1 -> Max/2
  Max/1 -> Divide1/1
  VehSpd/1 -> Abs/1
  Abs/1 -> Max/1
  Switch/1 -> Product2/2
  Constant1/1 -> Gain/1
  PwrLim/1 -> Switch/2
  Gain2/1 -> Switch/1
  Gain/1 -> Switch/3, Gain2/1

== system ZT_VehCtrl_18B_CAN/VehCtrl/MontionControl/VehTrqForward ==
  VehSpd : Inport
  VehDrv : Inport  Port=2
  PwrLim : Inport  Port=3
  Abs : Abs
  Constant : Constant  Value=VehTrqMax
  Constant1 : Constant  Value=VehPwrMax
  Constant2 : Constant  Value=WhlRadius
  Constant3 : Constant  Value=0.1  OutDataTypeStr=single
  Divide : Product  Inputs=*/
  Divide1 : Product  Inputs=*/
  Gain : Gain  Gain=1000
  Gain1 : Gain  Gain=0.01
  Gain2 : Gain  Gain=PwrLimFactor
  Max : MinMax  Function=max  Inputs=2
  Min : MinMax  Inputs=2
  Product : Product
  Product1 : Product
  Product2 : Product
  Switch : Switch  Criteria=u2 > Threshold
  VehTrq : Outport
  wires:
  Gain2/1 -> Switch/1
  PwrLim/1 -> Switch/2
  Constant1/1 -> Gain/1
  Switch/1 -> Product2/2
  Abs/1 -> Max/1
  VehSpd/1 -> Abs/1
  Max/1 -> Divide1/1
  Constant3/1 -> Max/2
  Constant2/1 -> Divide1/2
  Min/1 -> VehTrq/1
  Divide/1 -> Min/2
  Product/1 -> Product2/1
  Divide1/1 -> Divide/2
  Product2/1 -> Divide/1
  Gain1/1 -> Product/1, Product/2, Product1/1
  Product1/1 -> Min/1
  VehDrv/1 -> Gain1/1
  Gain/1 -> Gain2/1, Switch/3
  Constant/1 -> Product1/2

== system ZT_VehCtrl_18B_CAN/Initialization & SPI timer1/CS1 LS/Subsystem/SPI_en ==
  Action Port : ActionPort
  Add : Sum
  Add1 : Sum  Inputs=+++
  Constant1 : Constant  Value=0
  Constant11 : Constant  OutDataTypeStr=uint8
  Constant2 : Constant  OutDataTypeStr=uint8
  Constant3 : Constant  Value=0
  Constant9 : Constant  Value=128  OutDataTypeStr=uint8
  Data Type Conversion : DataTypeConversion
  Data Type Conversion1 : DataTypeConversion
  Gain : Gain  Gain=64
  Out1 : Outport
  Out2 : Outport  Port=2
  wires:
  Constant1/1 -> Add/1
  Constant9/1 -> Add1/1
  Add1/1 -> Data Type Conversion/1
  Constant11/1 -> Add1/2
  Constant2/1 -> Gain/1
  Gain/1 -> Add1/3
  Add/1 -> Data Type Conversion1/1
  Constant3/1 -> Add/2
  Data Type Conversion/1 -> Out1/1
  Data Type Conversion1/1 -> Out2/1

== system ZT_VehCtrl_18B_CAN/Initialization & SPI timer1/CS1 LS/Subsystem/clear  ==
  Action Port : ActionPort
  Add : Sum
  Add1 : Sum  Inputs=+++
  Constant1 : Constant
  Constant11 : Constant  Value=7  OutDataTypeStr=uint8
  Constant2 : Constant  Value=0  OutDataTypeStr=uint8
  Constant3 : Constant  Value=0
  Constant9 : Constant  Value=128  OutDataTypeStr=uint8
  Data Type Conversion : DataTypeConversion
  Data Type Conversion1 : DataTypeConversion
  Gain : Gain  Gain=64
  Out1 : Outport
  Out2 : Outport  Port=2
  wires:
  Constant3/1 -> Add/2
  Add/1 -> Data Type Conversion1/1
  Gain/1 -> Add1/3
  Constant2/1 -> Gain/1
  Constant11/1 -> Add1/2
  Add1/1 -> Data Type Conversion/1
  Data Type Conversion1/1 -> Out2/1
  Data Type Conversion/1 -> Out1/1
  Constant9/1 -> Add1/1
  Constant1/1 -> Add/1

== system ZT_VehCtrl_18B_CAN/Initialization & SPI timer1/CS1 LS/Subsystem/confi_enbit ==
  Action Port : ActionPort
  Add : Sum
  Add1 : Sum  Inputs=+++
  Constant1 : Constant
  Constant11 : Constant  Value=7  OutDataTypeStr=uint8
  Constant2 : Constant  OutDataTypeStr=uint8
  Constant3 : Constant  Value=128
  Constant9 : Constant  Value=128  OutDataTypeStr=uint8
  Data Type Conversion : DataTypeConversion
  Data Type Conversion1 : DataTypeConversion
  Gain : Gain  Gain=64
  Out1 : Outport
  Out2 : Outport  Port=2
  wires:
  Constant1/1 -> Add/1
  Constant9/1 -> Add1/1
  Add1/1 -> Data Type Conversion/1
  Constant11/1 -> Add1/2
  Constant2/1 -> Gain/1
  Gain/1 -> Add1/3
  Add/1 -> Data Type Conversion1/1
  Constant3/1 -> Add/2
  Data Type Conversion/1 -> Out1/1
  Data Type Conversion1/1 -> Out2/1

== system ZT_VehCtrl_18B_CAN/Initialization & SPI timer1/CS3 LS/Subsystem/A组配置 ==
  Action Port : ActionPort
  Add : Sum  Inputs=+++
  Add1 : Sum  Inputs=+++
  Bias : Bias  Bias=1
  Constant : Constant
  Constant10 : Constant  Value=2
  Constant9 : Constant  Value=80  OutDataTypeStr=uint8
  Data Store Read1 : DataStoreRead  DataStoreName=cnt2
  Data Store Write : DataStoreWrite  DataStoreName=SPI3_CTRL1
  Data Store Write1 : DataStoreWrite  DataStoreName=cnt2
  Data Type Conversion : DataTypeConversion  OutDataTypeStr=uint8
  Data Type Conversion1 : DataTypeConversion  OutDataTypeStr=uint8
  Data Type Conversion2 : DataTypeConversion
  Gain : Gain  Gain=4
  Gain1 : Gain
  Gain2 : Gain  Gain=4
  Gain3 : Gain
  Manual Switch : ManualSwitch  CurrentSetting=0
  PIN : Constant  Value=2
  SPI : Constant  Value=0
  Switch4 : Switch  Criteria=u2 > Threshold  Threshold=2
  default SPI : Constant  Value=0
  Out1 : Outport  VectorParamsAs1DForOutWhenUnconnected=on
  Out2 : Outport  Port=2  VectorParamsAs1DForOutWhenUnconnected=on
  wires:
  Switch4/1 -> Data Type Conversion2/1
  Constant/1 -> Switch4/3
  Constant10/1 -> Switch4/1
  Data Store Read1/1 -> Bias/1
  Bias/1 -> Data Store Write1/1, Switch4/2
  Data Type Conversion2/1 -> Data Store Write/1
  Data Type Conversion/1 -> Out1/1
  Data Type Conversion1/1 -> Out2/1
  Constant9/1 -> Add1/1
  Add/1 -> Data Type Conversion1/1
  [Mode] -> Gain3/1, Gain2/1, Gain1/1, Gain/1
  Gain2/1 -> Add/1
  Gain3/1 -> Add/2
  default SPI/1 -> Add/3
  Add1/1 -> Data Type Conversion/1
  Gain/1 -> Add1/2
  Gain1/1 -> Add1/3
  SPI/1 -> Manual Switch/1
  Manual Switch/1 -> [Mode]
  PIN/1 -> Manual Switch/2

== system ZT_VehCtrl_18B_CAN/Initialization & SPI timer1/CS3 LS/Subsystem/B组配置 ==
  Action Port : ActionPort
  Bias : Bias  Bias=1
  Constant : Constant  Value=2
  Constant1 : Constant  Value=0  OutDataTypeStr=uint8
  Constant10 : Constant  Value=3
  Constant9 : Constant  Value=96  OutDataTypeStr=uint8
  Data Store Read1 : DataStoreRead  DataStoreName=cnt2
  Data Store Write : DataStoreWrite  DataStoreName=SPI3_CTRL1
  Data Store Write1 : DataStoreWrite  DataStoreName=cnt2
  Data Type Conversion : DataTypeConversion  OutDataTypeStr=uint8
  Data Type Conversion1 : DataTypeConversion  OutDataTypeStr=uint8
  Data Type Conversion2 : DataTypeConversion
  Switch4 : Switch  Criteria=u2 > Threshold  Threshold=4
  Out1 : Outport  VectorParamsAs1DForOutWhenUnconnected=on
  Out2 : Outport  Port=2  VectorParamsAs1DForOutWhenUnconnected=on
  wires:
  Data Type Conversion2/1 -> Data Store Write/1
  Bias/1 -> Switch4/2, Data Store Write1/1
  Data Store Read1/1 -> Bias/1
  Constant10/1 -> Switch4/1
  Constant/1 -> Switch4/3
  Switch4/1 -> Data Type Conversion2/1
  Constant1/1 -> Data Type Conversion1/1
  Data Type Conversion/1 -> Out1/1
  Constant9/1 -> Data Type Conversion/1
  Data Type Conversion1/1 -> Out2/1

== system ZT_VehCtrl_18B_CAN/Initialization & SPI timer1/CS5 LS/Subsystem/SPI_en ==
  Action Port : ActionPort
  Add : Sum
  Add1 : Sum  Inputs=+++
  Constant1 : Constant  Value=0
  Constant11 : Constant  OutDataTypeStr=uint8
  Constant2 : Constant  OutDataTypeStr=uint8
  Constant3 : Constant  Value=0
  Constant9 : Constant  Value=128  OutDataTypeStr=uint8
  Data Type Conversion : DataTypeConversion
  Data Type Conversion1 : DataTypeConversion
  Gain : Gain  Gain=64
  Out1 : Outport
  Out2 : Outport  Port=2
  wires:
  Constant1/1 -> Add/1
  Constant9/1 -> Add1/1
  Add1/1 -> Data Type Conversion/1
  Constant11/1 -> Add1/2
  Constant2/1 -> Gain/1
  Gain/1 -> Add1/3
  Add/1 -> Data Type Conversion1/1
  Constant3/1 -> Add/2
  Data Type Conversion/1 -> Out1/1
  Data Type Conversion1/1 -> Out2/1

== system ZT_VehCtrl_18B_CAN/Initialization & SPI timer1/CS5 LS/Subsystem/clear  ==
  Action Port : ActionPort
  Add : Sum
  Add1 : Sum  Inputs=+++
  Constant1 : Constant
  Constant11 : Constant  Value=7  OutDataTypeStr=uint8
  Constant2 : Constant  Value=0  OutDataTypeStr=uint8
  Constant3 : Constant  Value=0
  Constant9 : Constant  Value=128  OutDataTypeStr=uint8
  Data Type Conversion : DataTypeConversion
  Data Type Conversion1 : DataTypeConversion
  Gain : Gain  Gain=64
  Out1 : Outport
  Out2 : Outport  Port=2
  wires:
  Constant3/1 -> Add/2
  Add/1 -> Data Type Conversion1/1
  Gain/1 -> Add1/3
  Constant2/1 -> Gain/1
  Constant11/1 -> Add1/2
  Add1/1 -> Data Type Conversion/1
  Data Type Conversion1/1 -> Out2/1
  Data Type Conversion/1 -> Out1/1
  Constant9/1 -> Add1/1
  Constant1/1 -> Add/1

== system ZT_VehCtrl_18B_CAN/Initialization & SPI timer1/CS5 LS/Subsystem/confi_enbit ==
  Action Port : ActionPort
  Add : Sum
  Add1 : Sum  Inputs=+++
  Constant1 : Constant
  Constant11 : Constant  Value=7  OutDataTypeStr=uint8
  Constant2 : Constant  OutDataTypeStr=uint8
  Constant3 : Constant  Value=128
  Constant9 : Constant  Value=128  OutDataTypeStr=uint8
  Data Type Conversion : DataTypeConversion
  Data Type Conversion1 : DataTypeConversion
  Gain : Gain  Gain=64
  Out1 : Outport
  Out2 : Outport  Port=2
  wires:
  Constant1/1 -> Add/1
  Constant9/1 -> Add1/1
  Add1/1 -> Data Type Conversion/1
  Constant11/1 -> Add1/2
  Constant2/1 -> Gain/1
  Gain/1 -> Add1/3
  Add/1 -> Data Type Conversion1/1
  Constant3/1 -> Add/2
  Data Type Conversion/1 -> Out1/1
  Data Type Conversion1/1 -> Out2/1
